simulink model "generic_src"  (Simulink 10.3)
settings: Solver=ode45  StartTime=0.0  StopTime=inf  RelTol=1e-3  EnableMultiTasking=on
undefined symbols (not defined in the file or in its folder): Area_Front, Area_Rear, ay_max_off, ay_max_on, ay_per_mu_max_off, ay_per_mu_max_on, Brake_ratio, brake_valve_ctrl_kP, cat1mode1_higher, cat1mode1_lower, cat1mode2_higher, cat1mode2_lower, cat1mode3_higher, cat1mode3_lower, cat2mode1_higher, cat2mode1_lower, cat2mode2_higher, cat2mode2_lower, cat2mode3_higher, cat2mode3_lower, delta_vel, diff_lock_fac, diff_lock_off, diff_lock_on, ESP_ctrl_kD, ESP_ctrl_kI, ESP_ctrl_kP, ESP_ctrl_restore_kI, ESP_min_throttle_fac, f_ax, f_slip, g, higherlimit_highvel, higherlimit_lowvel, highervel_fac, highervelocity_fac, InitialConditionForIntegrator, limit_acc, limit_selectlow, limit_starting, limit_vdiff, locktime_throttle, lowerlimit_highvel, lowerlimit_lowvel, lowervel_fac, lowervelocity_fac, min_throttle, MPS2KMPH, MSR_ctrl_kD, MSR_ctrl_kI, MSR_ctrl_kP, MSR_min_throttle_fac, PID_kP_sideslip, PID_kP_yawrate, RADpS2RpM, rBrake, RpM2RADpS, SH_SL_switch, sideslip_vel_corr, sidesplip_deviation_max ... (+35)
libraries: CarMaker4SL x136, simulink x55, simulink_extras x6
(part 1 of 9)
settings Model: Creator=IPG  LastModifiedBy=IPG  MultithreadedSim=on  ExtModeAutoUpdateStatusClock=off
settings DataIOCC: LimitDataPoints=on  SignalLoggingName=sigsOut
settings OptimizationCC: BooleanDataType=off  InitFltsAndDblsToZero=on
settings DebuggingCC: SaveWithParameterizedLinksMsg=none  SignalResolutionControl=TryResolveAllWithWarning  MultiTaskDSMMsg=warning  MultiTaskCondExecSysMsg=none  SFExecutionAtInitializationDiag=warning
settings HardwareCC: TargetUnknown=on
settings CodeAppCC: MaxIdLength=63
settings GRTTargetCC: TargetFcnLib=ansi_tfl_tmw.mat

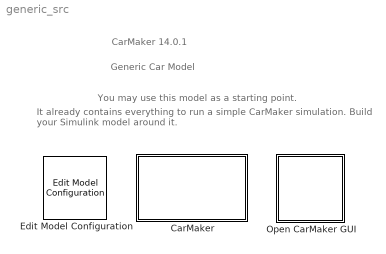
== system generic_src ==
  note: Generic Car Model
  note: You may use this model as a starting point.
  note: It already contains everything to run a simple CarMaker simulation.
      | Build your Simulink model around it.
  note: CarMaker 14.0.1
  CarMaker : Subsystem  TreatAsAtomicUnit=on
      mask Display: image(imread('CarMakerSys.png'));
  Edit Model Configuration : CarMaker4SL/Edit Model Configuration  SFunctionModules=''
  Open CarMaker GUI : Subsystem  LoadFcn=if ~length(which('cmself')), cmenv; end
      settings: OpenFcn=cmblockmagic('gui_fix_display'); CM_Simulink
      mask Display: image(imread('CarMakerGUI.png'));

== system generic_src/CarMaker ==
  CM_FIRST : Subsystem
  CM_LAST : Subsystem
  DrivMan : Subsystem
  Ground : Ground
  IPG Vehicle : Subsystem
  Terminator : Terminator
  VehicleControl : Subsystem
  wires:
  DrivMan/2(DrivMan.Out) -> VehicleControl/2(DrivMan.In)
  DrivMan/1(Sync_Out) -> VehicleControl/1(Sync_In)
  CM_FIRST/2(Env.Misc) -> DrivMan/2(Env.Misc)
  CM_FIRST/1(Sync_Out) -> DrivMan/1(Sync_In)
  CM_LAST/1(Sync_Out) -> Terminator/1
  Ground/1 -> CM_FIRST/1(Sync_In)
  IPG Vehicle/1(Sync_Out) -> CM_LAST/1(Sync_In)
  VehicleControl/1(Sync_Out) -> IPG Vehicle/1(Sync_In)
  VehicleControl/3(VhclCtrl.Steering) -> IPG Vehicle/3(VhclCtrl.Steering)
  VehicleControl/4(Vhcl.Wheel.In) -> IPG Vehicle/4(Vhcl.Wheel.In)
  VehicleControl/5(Vhcl.Misc) -> IPG Vehicle/5(Vhcl.Misc)
  VehicleControl/6(VhclCtrl.Brake) -> IPG Vehicle/6(VhclCtrl.Brake)
  VehicleControl/7(VhclCtrl.PT) -> IPG Vehicle/7(VhclCtrl.PT)
  VehicleControl/2(Vhcl.Model.Source) -> IPG Vehicle/2(Vhcl.Model.Source)

== system generic_src/Open CarMaker GUI ==
  S-Function : S-Function  FunctionName=cm_gui  SFunctionDeploymentMode=off  EnableBusSupport=off

== system generic_src/CarMaker/CM_FIRST ==
  Sync_In : Inport
  BusCreator1 : BusCreator  Inputs=8
  BusCreator2 : BusCreator  Inputs=6
  Demux1 : Demux  Outputs=14
      settings: DisplayOption=none
  Environment : S-Function  FunctionName=CM_Sfun  Parameters='Environment'  SFunctionDeploymentMode=off  EnableBusSupport=off
  IoIn : S-Function  FunctionName=CM_Sfun  Parameters='IoIn'  SFunctionDeploymentMode=off  EnableBusSupport=off
  Terminator : Terminator
  Sync_Out : Outport  VectorParamsAs1DForOutWhenUnconnected=off
  Env.Misc : Outport  Port=2  VectorParamsAs1DForOutWhenUnconnected=off
  wires:
  BusCreator2/1 -> Terminator/1  "IF Environment (in)"
  BusCreator1/1 -> Env.Misc/1
  Demux1/14 -> BusCreator2/6  "Env sRoad"
  Demux1/13 -> BusCreator2/5  "Env PoI_GCS Elev"
  Demux1/12 -> BusCreator2/4  "Env PoI_GCS Lat"
  Demux1/11 -> BusCreator2/3  "Env PoI_GCS Long"
  Demux1/10 -> BusCreator2/2  "Env Time"
  Demux1/9 -> BusCreator2/1  "Env yDay"
  Demux1/8 -> BusCreator1/8  "Env WindVel_tot z"
  Demux1/7 -> BusCreator1/7  "Env WindVel_tot y"
  Demux1/6 -> BusCreator1/6  "Env WindVel_tot x"
  Demux1/5 -> BusCreator1/5  "Env SolarRadiation"
  Demux1/4 -> BusCreator1/4  "Env AirHumidity"
  Demux1/3 -> BusCreator1/3  "Env AirPressure"
  Demux1/2 -> BusCreator1/2  "Env AirDensity"
  Demux1/1 -> BusCreator1/1  "Env Temperature"
  Environment/2 -> Demux1/1
  Environment/1 -> Sync_Out/1
  IoIn/1 -> Environment/1
  Sync_In/1 -> IoIn/1

== system generic_src/CarMaker/CM_LAST ==
  Sync_In : Inport
  CM_User : S-Function  FunctionName=CM_Sfun  Parameters='CM_User'  SFunctionDeploymentMode=off  EnableBusSupport=off
  IoOut : S-Function  FunctionName=CM_Sfun  Parameters='IoOut'  SFunctionDeploymentMode=off  EnableBusSupport=off
  Sync_Out : Outport  VectorParamsAs1DForOutWhenUnconnected=off
  wires:
  IoOut/1 -> Sync_Out/1
  CM_User/1 -> IoOut/1
  Sync_In/1 -> CM_User/1

== system generic_src/CarMaker/DrivMan ==
  note: There's rarely a reason to override DrivMan signals.
      | Use the VehicleControl interface for this purpose.
  Sync_In : Inport
  Env.Misc : Inport  Port=2
  BusCreator : BusCreator  Inputs=20
  Demux : Demux  Outputs=20
      settings: DisplayOption=none
  DrivMan : S-Function  FunctionName=CM_Sfun  Parameters='DrivMan'  SFunctionDeploymentMode=off  EnableBusSupport=off
  Ground : Ground
  Ground1 : Ground
  Ground2 : Ground
  Terminator : Terminator
  Terminator1 : Terminator
  Terminator2 : Terminator
  Sync_Out : Outport  VectorParamsAs1DForOutWhenUnconnected=off
  DrivMan.Out : Outport  Port=2  VectorParamsAs1DForOutWhenUnconnected=off
  wires:
  Demux/20 -> BusCreator/20  "DrivMan Steering Trq"
  Demux/19 -> BusCreator/19  "DrivMan Steering AngAcc"
  Demux/18 -> BusCreator/18  "DrivMan Steering AngVel"
  Demux/17 -> BusCreator/17  "DrivMan Steering Ang"
  Demux/16 -> BusCreator/16  "DrivMan Gas"
  Demux/15 -> BusCreator/15  "DrivMan Clutch"
  Demux/14 -> BusCreator/14  "DrivMan BrakePark"
  Demux/13 -> BusCreator/13  "DrivMan Brake"
  Demux/12 -> BusCreator/12  "DrivMan GearNo"
  Demux/8 -> BusCreator/8  "DrivMan SelectorCtrl"
  Demux/7 -> BusCreator/7  "DrivMan UserSignal4"
  Demux/6 -> BusCreator/6  "DrivMan UserSignal3"
  Demux/5 -> BusCreator/5  "DrivMan UserSignal2"
  Demux/4 -> BusCreator/4  "DrivMan UserSignal1"
  Demux/3 -> BusCreator/3  "DrivMan UserSignal0"
  Demux/2 -> BusCreator/2  "DrivMan Key"
  Env.Misc/1 -> DrivMan/2
  Sync_In/1 -> DrivMan/1
  DrivMan/1 -> Sync_Out/1
  BusCreator/1 -> DrivMan.Out/1
  DrivMan/2 -> Demux/1
  Demux/1 -> BusCreator/1  "DrivMan SST"
  Demux/9 -> Terminator/1  "DrivMan DigitalSelectorCtrl0"
  Demux/10 -> Terminator1/1  "DrivMan DigitalSelectorCtrl1"
  Demux/11 -> Terminator2/1  "DrivMan DigitalSelectorCtrl2"
  Ground/1 -> BusCreator/9
  Ground1/1 -> BusCreator/10
  Ground2/1 -> BusCreator/11

== system generic_src/CarMaker/IPG Vehicle ==
  Sync_In : Inport
  Vhcl.Model.Source : Inport  Port=2
  VhclCtrl.Steering : Inport  Port=3
  Vhcl.Wheel.In : Inport  Port=4
  Vhcl.Misc : Inport  Port=5
  VhclCtrl.Brake : Inport  Port=6
  VhclCtrl.PT : Inport  Port=7
  Brake : Subsystem
  CarAndTrailer : Subsystem
  PowerTrain : Subsystem
  Stop Simulation : Stop
  VehicleSource_BuiltIn : simulink/Logic and Bit Operations/Compare To Constant  relop=~=  const=1  OutDataTypeStr=boolean  ZeroCross=off
  Sync_Out : Outport  VectorParamsAs1DForOutWhenUnconnected=off
  wires:
  VhclCtrl.PT/1 -> PowerTrain/3(VhclCtrl.PT)
  Brake/1(Sync_Out) -> PowerTrain/1(Sync_In)
  CarAndTrailer/1(Sync_Out) -> Brake/1(Sync_In)
  CarAndTrailer/2(Brake.IF.In) -> Brake/2(Brake.IF.In)
  VhclCtrl.Brake/1 -> Brake/3(VhclCtrl.Brake)
  PowerTrain/1(Sync_Out) -> Sync_Out/1
  Vhcl.Misc/1 -> CarAndTrailer/4(Vhcl.Misc)
  Vhcl.Wheel.In/1 -> CarAndTrailer/3(Vhcl.Wheel.In)
  VhclCtrl.Steering/1 -> CarAndTrailer/2(VhclCtrl.Steering)
  Sync_In/1 -> CarAndTrailer/1(Sync_In)
  Vhcl.Model.Source/1 -> VehicleSource_BuiltIn/1
  VehicleSource_BuiltIn/1 -> Stop Simulation/1
  Brake/2(Vhcl.Wheel.PT) -> PowerTrain/2(Vhcl.Wheel.PT)

== system generic_src/CarMaker/VehicleControl ==
  note: <Your model here>
  note: When implementing a vehicle control model,
      | be sure to add '-disablevehiclecontrol' to the command line arguments
      | in the CarMaker Model Configuration block.
      | Otherwise your model will possibly not see the original DrivMan signals
      | on its inputs, but those of a currently activated C-coded vehicle control model instead.
  Sync_In : Inport
  DrivMan.In : Inport  Port=2
  Bus Creator2 : BusCreator  Inputs=2
  CreateBus Vhcl.Misc : Subsystem
  CreateBus Vhcl.Wheel.In : Subsystem
  CreateBus VhclCtrl : Subsystem
  CreateBus VhclCtrl.PT : Subsystem
  CreateBus VhclCtrl.Steering : Subsystem
  Demux2 : Demux  Outputs=2
      settings: DisplayOption=none
  VehicleControl : S-Function  FunctionName=CM_Sfun  Parameters='VehicleControl'  SFunctionDeploymentMode=off  EnableBusSupport=off
  VehicleControlUpd : S-Function  FunctionName=CM_Sfun  Parameters='VehicleControlUpd'  SFunctionDeploymentMode=off  EnableBusSupport=off
  Sync_Out : Outport  VectorParamsAs1DForOutWhenUnconnected=off
  Vhcl.Model.Source : Outport  Port=2  VectorParamsAs1DForOutWhenUnconnected=off
  VhclCtrl.Steering : Outport  Port=3  VectorParamsAs1DForOutWhenUnconnected=off
  Vhcl.Wheel.In : Outport  Port=4  VectorParamsAs1DForOutWhenUnconnected=off
  Vhcl.Misc : Outport  Port=5  VectorParamsAs1DForOutWhenUnconnected=off
  VhclCtrl.Brake : Outport  Port=6  VectorParamsAs1DForOutWhenUnconnected=off
  VhclCtrl.PT : Outport  Port=7  VectorParamsAs1DForOutWhenUnconnected=off
  wires:
  CreateBus VhclCtrl/1(Out) -> VehicleControlUpd/2
  VehicleControl/2 -> CreateBus VhclCtrl/1(In)
  VehicleControlUpd/2 -> Vhcl.Model.Source/1
  VehicleControlUpd/4 -> CreateBus Vhcl.Wheel.In/1(In1)
  VehicleControlUpd/5 -> CreateBus Vhcl.Misc/1(In1)
  VehicleControlUpd/6 -> Demux2/1
  VehicleControlUpd/7 -> CreateBus VhclCtrl.PT/1(In1)
  VehicleControlUpd/3 -> CreateBus VhclCtrl.Steering/1(In1)
  CreateBus Vhcl.Misc/1(Out1) -> Vhcl.Misc/1
  CreateBus Vhcl.Wheel.In/1(Out1) -> Vhcl.Wheel.In/1
  DrivMan.In/1 -> VehicleControl/2
  VehicleControl/1 -> VehicleControlUpd/1
  Sync_In/1 -> VehicleControl/1
  CreateBus VhclCtrl.PT/1(Out1) -> VhclCtrl.PT/1
  Bus Creator2/1 -> VhclCtrl.Brake/1
  CreateBus VhclCtrl.Steering/1(Out1) -> VhclCtrl.Steering/1
  VehicleControlUpd/1 -> Sync_Out/1
  Demux2/2 -> Bus Creator2/2  "VhclCtrl BrakePark"
  Demux2/1 -> Bus Creator2/1  "VhclCtrl Brake"

== system generic_src/CarMaker/IPG Vehicle/Brake ==
  note: When replacing the entire braking system,
      | be sure to disable the IPG brake model by using the brake
      | model 'Model Manager off' in the vehicle GUI.
  note: <Your model here>
  Sync_In : Inport
  Brake.IF.In : Inport  Port=2
  VhclCtrl.Brake : Inport  Port=3
  Brake : S-Function  FunctionName=CM_Sfun  Parameters='Brake'  SFunctionDeploymentMode=off  EnableBusSupport=off
  BrakeUpd : S-Function  FunctionName=CM_Sfun  Parameters='BrakeUpd'  SFunctionDeploymentMode=off  EnableBusSupport=off
  BusCreator1 : BusCreator  Inputs=16
  CreateBus Vhcl.Wheel.PT : Subsystem
  Demux : Demux  Outputs=16
      settings: DisplayOption=none
  HydBrakeCU Example : Subsystem
  Sync_Out : Outport  VectorParamsAs1DForOutWhenUnconnected=off
  Vhcl.Wheel.PT : Outport  Port=2  VectorParamsAs1DForOutWhenUnconnected=off
  wires:
  Demux/16 -> BusCreator1/16  "Brake IF Trq_DriveSrc_trg d3"
  Demux/15 -> BusCreator1/15  "Brake IF Trq_DriveSrc_trg d2"
  Demux/14 -> BusCreator1/14  "Brake IF Trq_DriveSrc_trg d1"
  Demux/13 -> BusCreator1/13  "Brake IF Trq_DriveSrc_trg d0"
  Demux/12 -> BusCreator1/12  "Brake IF Trq_Reg_trg RR"
  Demux/11 -> BusCreator1/11  "Brake IF Trq_Reg_trg RL"
  Demux/10 -> BusCreator1/10  "Brake IF Trq_Reg_trg FR"
  Demux/9 -> BusCreator1/9  "Brake IF Trq_Reg_trg FL"
  Demux/8 -> BusCreator1/8  "Brake IF Trq_PB RR"
  Demux/7 -> BusCreator1/7  "Brake IF Trq_PB RL"
  Demux/6 -> BusCreator1/6  "Brake IF Trq_PB FR"
  Demux/5 -> BusCreator1/5  "Brake IF Trq_PB FL"
  Demux/4 -> BusCreator1/4  "Brake IF Trq_WB RR"
  Demux/3 -> BusCreator1/3  "Brake IF Trq_WB RL"
  Demux/2 -> BusCreator1/2  "Brake IF Trq_WB FR"
  Demux/1 -> BusCreator1/1  "Brake IF Trq_WB FL"
  Brake/2 -> Demux/1
  BusCreator1/1 -> BrakeUpd/2
  BrakeUpd/1 -> Sync_Out/1
  Brake/1 -> BrakeUpd/1  "Sync"
  Brake.IF.In/1 -> Brake/2
  VhclCtrl.Brake/1 -> Brake/3
  Sync_In/1 -> Brake/1
  BrakeUpd/2 -> CreateBus Vhcl.Wheel.PT/1(In)
  CreateBus Vhcl.Wheel.PT/1(Out) -> Vhcl.Wheel.PT/1

== system generic_src/CarMaker/IPG Vehicle/CarAndTrailer ==
  Sync_In : Inport
  VhclCtrl.Steering : Inport  Port=2
  Vhcl.Wheel.In : Inport  Port=3
  Vhcl.Misc : Inport  Port=4
  CarAndTrailerUpd : Subsystem
  Forces : Subsystem
  Ground : Ground
  Kinematics : Subsystem
  Kinetics : Subsystem
  Steering : Subsystem
  Terminator : Terminator
  Terminator1 : Terminator
  Trailer : Subsystem
  Sync_Out : Outport  VectorParamsAs1DForOutWhenUnconnected=off
  Brake.IF.In : Outport  Port=2  VectorParamsAs1DForOutWhenUnconnected=off
  wires:
  Trailer/9(Car.Hitch.FrcTrq) -> CarAndTrailerUpd/9(Car.Hitch.FrcTrq)
  Trailer/8(Vhcl.Wheel.RR) -> CarAndTrailerUpd/8(Vhcl.Wheel.RR)
  Trailer/7(Vhcl.Wheel.RL) -> CarAndTrailerUpd/7(Vhcl.Wheel.RL)
  Trailer/6(Vhcl.Wheel.FR) -> CarAndTrailerUpd/6(Vhcl.Wheel.FR)
  Trailer/5(Vhcl.Wheel.FL) -> CarAndTrailerUpd/5(Vhcl.Wheel.FL)
  Trailer/4(Vhcl.PoI) -> CarAndTrailerUpd/4(Vhcl.PoI)
  Trailer/3(Vhcl.Motion) -> CarAndTrailerUpd/3(Vhcl.Motion)
  Trailer/2(Vhcl.Steering) -> CarAndTrailerUpd/2(Vhcl.Steering)
  Trailer/1(Sync_Out) -> CarAndTrailerUpd/1(Sync_In)
  CarAndTrailerUpd/2(Brake.IF.In) -> Brake.IF.In/1
  CarAndTrailerUpd/1(Sync_Out) -> Sync_Out/1
  Vhcl.Misc/1 -> Terminator1/1
  Vhcl.Wheel.In/1 -> Terminator/1
  Kinetics/6(WheelCarrier.Misc) -> Trailer/6(WheelCarrier.Misc)
  Kinetics/5(Car.Trq_T2W) -> Trailer/5(Car.Trq_T2W)
  Steering/2(Steer.IF) -> ?
  Kinetics/4(Car.Fr1) -> Trailer/4(Car.Fr1)
  Kinetics/3(Car.Hitch) -> Trailer/3(Car.Hitch)
  Kinetics/2(Trailer.Load) -> Trailer/2(Trailer.Load)
  VhclCtrl.Steering/1 -> Steering/2(VhclCtrl.Steering)
  Sync_In/1 -> Steering/1(Sync_In)
  Steering/1(Sync_Out) -> ?
  Kinetics/1(Sync_Out) -> Trailer/1(Sync_In)
  Ground/1 -> CarAndTrailerUpd/10(Vhcl.Fr1A)
  ? -> ?
  ? -> ?
  ? -> ?
  Forces/8(TireRR_Out) -> ?
  Forces/7(TireRL_Out) -> ?
  Forces/6(TireFR_Out) -> ?
  Forces/5(TireFL_Out) -> ?
  Forces/4(Car.Load) -> ?
  Forces/2(Car.Virtual) -> ?
  ? -> Forces/6(lSpring)
  ? -> Forces/7(vDamp)
  Forces/3(Car.Aero) -> ?
  Forces/1(Sync_Out) -> ?
  ? -> Forces/5(TireRR_In)
  ? -> Forces/4(TireRL_In)
  ? -> Forces/3(TireFR_In)
  ? -> Forces/2(TireFL_In)
  ? -> Forces/1(Sync_In)
  ? -> Forces/8(lStabi)
  ? -> ?
  ? -> Forces/9(lBuf)

== system generic_src/CarMaker/IPG Vehicle/PowerTrain ==
  note: When replacing the entire powertrain,
      | be sure to disable the IPG powertrain model by using the powertrain
      | model 'Model Manager off' in the vehicle GUI.
  note: <Your model here>
  Sync_In : Inport
  Vhcl.Wheel.PT : Inport  Port=2
  VhclCtrl.PT : Inport  Port=3
  BusCreator1 : BusCreator  Inputs=42
  Demux1 : Demux  Outputs=42
      settings: DisplayOption=none
  Ground : Ground
  MCU Example : Subsystem
  PTControl Example : Subsystem
  PowerTrain : S-Function  FunctionName=CM_Sfun  Parameters='PowerTrain'  SFunctionDeploymentMode=off  EnableBusSupport=off
  PowerTrainUpd : S-Function  FunctionName=CM_Sfun  Parameters='PowerTrainUpd'  SFunctionDeploymentMode=off  EnableBusSupport=off
  Sync_Out : Outport  VectorParamsAs1DForOutWhenUnconnected=off
  wires:
  BusCreator1/1 -> PowerTrainUpd/2
  Demux1/42 -> BusCreator1/42  "PT IF WRR Trq_BrakeReg_max"
  Demux1/41 -> BusCreator1/41  "PT IF WRR Trq_BrakeReg"
  Demux1/40 -> BusCreator1/40  "PT IF WRR Trq_Supp2WC"
  Demux1/39 -> BusCreator1/39  "PT IF WRR Trq_Drive"
  Demux1/38 -> BusCreator1/38  "PT IF WRR Trq_B2W"
  Demux1/37 -> BusCreator1/37  "PT IF WRR rotv"
  Demux1/36 -> BusCreator1/36  "PT IF WRR rot"
  Demux1/35 -> BusCreator1/35  "PT IF WRL Trq_BrakeReg_max"
  Demux1/34 -> BusCreator1/34  "PT IF WRL Trq_BrakeReg"
  Demux1/33 -> BusCreator1/33  "PT IF WRL Trq_Supp2WC"
  Demux1/32 -> BusCreator1/32  "PT IF WRL Trq_Drive"
  Demux1/31 -> BusCreator1/31  "PT IF WRL Trq_B2W"
  Demux1/30 -> BusCreator1/30  "PT IF WRL rotv"
  Demux1/29 -> BusCreator1/29  "PT IF WRL rot"
  Demux1/28 -> BusCreator1/28  "PT IF WFR Trq_BrakeReg_max"
  Demux1/27 -> BusCreator1/27  "PT IF WFR Trq_BrakeReg"
  Demux1/26 -> BusCreator1/26  "PT IF WFR Trq_Supp2WC"
  Demux1/25 -> BusCreator1/25  "PT IF WFR Trq_Drive"
  Demux1/24 -> BusCreator1/24  "PT IF WFR Trq_B2W"
  Demux1/23 -> BusCreator1/23  "PT IF WFR rotv"
  Demux1/22 -> BusCreator1/22  "PT IF WFR rot"
  Demux1/21 -> BusCreator1/21  "PT IF WFL Trq_BrakeReg_max"
  Demux1/20 -> BusCreator1/20  "PT IF WFL Trq_BrakeReg"
  Demux1/19 -> BusCreator1/19  "PT IF WFL Trq_Supp2WC"
  Demux1/18 -> BusCreator1/18  "PT IF WFL Trq_Drive"
  Demux1/17 -> BusCreator1/17  "PT IF WFL Trq_B2W"
  Demux1/16 -> BusCreator1/16  "PT IF WFL rotv"
  Demux1/15 -> BusCreator1/15  "PT IF WFL rot"
  Demux1/14 -> BusCreator1/14  "PT IF DL_iDiff_mean"
  Demux1/13 -> BusCreator1/13  "PT IF Trq_Supp2BdyEng y"
  Demux1/12 -> BusCreator1/12  "PT IF Trq_Supp2BdyEng x"
  Demux1/11 -> BusCreator1/11  "PT IF Trq_Supp2Bdy1B z"
  Demux1/10 -> BusCreator1/10  "PT IF Trq_Supp2Bdy1B y"
  Demux1/9 -> BusCreator1/9  "PT IF Trq_Supp2Bdy1B x"
  Demux1/8 -> BusCreator1/8  "PT IF Trq_Supp2Bdy1 z"
  Demux1/7 -> BusCreator1/7  "PT IF Trq_Supp2Bdy1 y"
  Demux1/6 -> BusCreator1/6  "PT IF Trq_Supp2Bdy1 x"
  Demux1/5 -> BusCreator1/5  "PT IF Engine_rotv"
  Demux1/4 -> BusCreator1/4  "PT IF GearNo"
  Demux1/3 -> BusCreator1/3  "PT IF OperationError"
  Demux1/2 -> BusCreator1/2  "PT IF OperationState"
  Demux1/1 -> BusCreator1/1  "PT IF Ignition"
  Sync_In/1 -> PowerTrain/1
  PowerTrain/2 -> Demux1/1
  PowerTrainUpd/1 -> Sync_Out/1
  PowerTrain/1 -> PowerTrainUpd/1  "Sync"
  VhclCtrl.PT/1 -> PowerTrain/3
  Vhcl.Wheel.PT/1 -> PowerTrain/2
  Ground/1 -> PTControl Example/1(Sync_In), MCU Example/1(Sync_In), PTControl Example/2(VhclCtrl.PT)

== system generic_src/CarMaker/VehicleControl/CreateBus Vhcl.Misc ==
  In1 : Inport
  BusCreator : BusCreator  Inputs=11
  Demux : Demux  Outputs=11
      settings: DisplayOption=none
  Out1 : Outport  VectorParamsAs1DForOutWhenUnconnected=off
  wires:
  Demux/11 -> BusCreator/11  "Vhcl Wind_vel_0 z"
  Demux/10 -> BusCreator/10  "Vhcl Wind_vel_0 y"
  Demux/9 -> BusCreator/9  "Vhcl Wind_vel_0 x"
  Demux/8 -> BusCreator/8  "Vhcl Trq_DL2BdyEng y"
  Demux/7 -> BusCreator/7  "Vhcl Trq_DL2BdyEng x"
  Demux/6 -> BusCreator/6  "Vhcl Trq_DL2Bdy1B z"
  Demux/5 -> BusCreator/5  "Vhcl Trq_DL2Bdy1B y"
  Demux/4 -> BusCreator/4  "Vhcl Trq_DL2Bdy1B x"
  Demux/3 -> BusCreator/3  "Vhcl Trq_DL2Bdy1 z"
  Demux/2 -> BusCreator/2  "Vhcl Trq_DL2Bdy1 y"
  Demux/1 -> BusCreator/1  "Vhcl Trq_DL2Bdy1 x"
  In1/1 -> Demux/1
  BusCreator/1 -> Out1/1

== system generic_src/CarMaker/VehicleControl/CreateBus Vhcl.Wheel.In ==
  In1 : Inport
  Bus Creator1 : BusCreator  Inputs=12
  Demux1 : Demux  Outputs=12
      settings: DisplayOption=none
  Out1 : Outport  VectorParamsAs1DForOutWhenUnconnected=off
  wires:
  Demux1/12 -> Bus Creator1/12  "Vhcl Wheel RR rotv"
  Demux1/11 -> Bus Creator1/11  "Vhcl Wheel RR Trq_DL2WC"
  Demux1/10 -> Bus Creator1/10  "Vhcl Wheel RR Trq_B2WC"
  Demux1/9 -> Bus Creator1/9  "Vhcl Wheel RL rotv"
  Demux1/8 -> Bus Creator1/8  "Vhcl Wheel RL Trq_DL2WC"
  Demux1/7 -> Bus Creator1/7  "Vhcl Wheel RL Trq_B2WC"
  Demux1/6 -> Bus Creator1/6  "Vhcl Wheel FR rotv"
  Demux1/5 -> Bus Creator1/5  "Vhcl Wheel FR Trq_DL2WC"
  Demux1/4 -> Bus Creator1/4  "Vhcl Wheel FR Trq_B2WC"
  Demux1/3 -> Bus Creator1/3  "Vhcl Wheel FL rotv"
  In1/1 -> Demux1/1
  Bus Creator1/1 -> Out1/1
  Demux1/2 -> Bus Creator1/2  "Vhcl Wheel FL Trq_DL2WC"
  Demux1/1 -> Bus Creator1/1  "Vhcl Wheel FL Trq_B2WC"

== system generic_src/CarMaker/VehicleControl/CreateBus VhclCtrl ==
  In : Inport
  BusCreator : BusCreator  Inputs=29
  Demux : Demux  Outputs=29
      settings: DisplayOption=none
  Out : Outport  VectorParamsAs1DForOutWhenUnconnected=off
  wires:
  In/1 -> Demux/1
  BusCreator/1 -> Out/1
  Demux/1 -> BusCreator/1  "VhclCtrl SST"
  Demux/2 -> BusCreator/2  "VhclCtrl Key"
  Demux/3 -> BusCreator/3  "VhclCtrl UserSignal0"
  Demux/4 -> BusCreator/4  "VhclCtrl UserSignal1"
  Demux/5 -> BusCreator/5  "VhclCtrl UserSignal2"
  Demux/6 -> BusCreator/6  "VhclCtrl UserSignal3"
  Demux/7 -> BusCreator/7  "VhclCtrl UserSignal4"
  Demux/8 -> BusCreator/8  "VhclCtrl GearNo"
  Demux/9 -> BusCreator/9  "VhclCtrl SelectorCtrl"
  Demux/10 -> BusCreator/10  "VhclCtrl Brake"
  Demux/11 -> BusCreator/11  "VhclCtrl BrakePark"
  Demux/12 -> BusCreator/12  "VhclCtrl Clutch"
  Demux/13 -> BusCreator/13  "VhclCtrl Gas"
  Demux/14 -> BusCreator/14  "VhclCtrl Steering Ang"
  Demux/15 -> BusCreator/15  "VhclCtrl Steering AngVel"
  Demux/16 -> BusCreator/16  "VhclCtrl Steering AngAcc"
  Demux/17 -> BusCreator/17  "VhclCtrl Steering Trq"
  Demux/18 -> BusCreator/18  "VhclCtrl Lights LowBeam"
  Demux/19 -> BusCreator/19  "VhclCtrl Lights HighBeam"
  Demux/20 -> BusCreator/20  "VhclCtrl Lights Daytime"
  Demux/21 -> BusCreator/21  "VhclCtrl Lights ParkL"
  Demux/22 -> BusCreator/22  "VhclCtrl Lights ParkR"
  Demux/23 -> BusCreator/23  "VhclCtrl Lights IndL"
  Demux/24 -> BusCreator/24  "VhclCtrl Lights IndR"
  Demux/25 -> BusCreator/25  "VhclCtrl Lights FogFrontL"
  Demux/26 -> BusCreator/26  "VhclCtrl Lights FogFrontR"
  Demux/27 -> BusCreator/27  "VhclCtrl Lights FogRear"
  Demux/28 -> BusCreator/28  "VhclCtrl Lights Brake"
  Demux/29 -> BusCreator/29  "VhclCtrl Lights Reverse"

== system generic_src/CarMaker/VehicleControl/CreateBus VhclCtrl.PT ==
  In1 : Inport
  BusCreator1 : BusCreator  Inputs=12
  Demux1 : Demux  Outputs=12
      settings: DisplayOption=none
  Out1 : Outport  VectorParamsAs1DForOutWhenUnconnected=off
  wires:
  Demux1/12 -> BusCreator1/12  "VhclCtrl Brake"
  Demux1/11 -> BusCreator1/11  "VhclCtrl Gas"
  Demux1/10 -> BusCreator1/10  "VhclCtrl Clutch"
  Demux1/9 -> BusCreator1/9  "VhclCtrl SelectorCtrl"
  Demux1/8 -> BusCreator1/8  "VhclCtrl GearNo"
  Demux1/7 -> BusCreator1/7  "VhclCtrl UserSignal4"
  Demux1/6 -> BusCreator1/6  "VhclCtrl UserSignal3"
  Demux1/5 -> BusCreator1/5  "VhclCtrl UserSignal2"
  Demux1/4 -> BusCreator1/4  "VhclCtrl UserSignal1"
  Demux1/3 -> BusCreator1/3  "VhclCtrl UserSignal0"
  Demux1/2 -> BusCreator1/2  "VhclCtrl Key"
  Demux1/1 -> BusCreator1/1  "VhclCtrl SST"
  In1/1 -> Demux1/1
  BusCreator1/1 -> Out1/1

== system generic_src/CarMaker/VehicleControl/CreateBus VhclCtrl.Steering ==
  In1 : Inport
  Bus Creator : BusCreator  Inputs=5
  Demux : Demux  Outputs=5
      settings: DisplayOption=none
  Out1 : Outport  VectorParamsAs1DForOutWhenUnconnected=off
  wires:
  In1/1 -> Demux/1
  Bus Creator/1 -> Out1/1
  Demux/1 -> Bus Creator/1  "VhclCtrl Steering Ang"
  Demux/5 -> Bus Creator/5  "VhclCtrl Steering SteerByTrq"
  Demux/3 -> Bus Creator/3  "VhclCtrl Steering AngAcc"
  Demux/2 -> Bus Creator/2  "VhclCtrl Steering AngVel"
  Demux/4 -> Bus Creator/4  "VhclCtrl Steering Trq"

== system generic_src/CarMaker/IPG Vehicle/Brake/CreateBus Vhcl.Wheel.PT ==
  In : Inport
  BusCreator1 : BusCreator  Inputs=20
  Demux1 : Demux  Outputs=20
      settings: DisplayOption=none
  Out : Outport  VectorParamsAs1DForOutWhenUnconnected=off
  wires:
  Demux1/20 -> BusCreator1/20  "Vhcl Trq_DriveSrc_trg d3"
  Demux1/19 -> BusCreator1/19  "Vhcl Trq_DriveSrc_trg d2"
  Demux1/18 -> BusCreator1/18  "Vhcl Trq_DriveSrc_trg d1"
  Demux1/17 -> BusCreator1/17  "Vhcl Trq_DriveSrc_trg d0"
  Demux1/16 -> BusCreator1/16  "Vhcl Wheel RR WhlBearing"
  Demux1/15 -> BusCreator1/15  "Vhcl Wheel RR Trq_T2W"
  Demux1/14 -> BusCreator1/14  "Vhcl Wheel RR Trq_BrakeReg_trg"
  Demux1/13 -> BusCreator1/13  "Vhcl Wheel RR Trq_Brake"
  Demux1/12 -> BusCreator1/12  "Vhcl Wheel RL WhlBearing"
  Demux1/11 -> BusCreator1/11  "Vhcl Wheel RL Trq_T2W"
  Demux1/10 -> BusCreator1/10  "Vhcl Wheel RL Trq_BrakeReg_trg"
  Demux1/9 -> BusCreator1/9  "Vhcl Wheel RL Trq_Brake"
  Demux1/8 -> BusCreator1/8  "Vhcl Wheel FR WhlBearing"
  Demux1/7 -> BusCreator1/7  "Vhcl Wheel FR Trq_T2W"
  Demux1/6 -> BusCreator1/6  "Vhcl Wheel FR Trq_BrakeReg_trg"
  Demux1/5 -> BusCreator1/5  "Vhcl Wheel FR Trq_Brake"
  Demux1/4 -> BusCreator1/4  "Vhcl Wheel FL WhlBearing"
  Demux1/3 -> BusCreator1/3  "Vhcl Wheel FL Trq_T2W"
  Demux1/2 -> BusCreator1/2  "Vhcl Wheel FL Trq_BrakeReg_trg"
  Demux1/1 -> BusCreator1/1  "Vhcl Wheel FL Trq_Brake"
  BusCreator1/1 -> Out/1
  In/1 -> Demux1/1

== system generic_src/CarMaker/IPG Vehicle/Brake/HydBrakeCU Example ==
  Sync_In : Inport
  Bus Assignment : BusAssignment  AssignedSignals=HydBrakeCU_Out Valve_FL_Inlet,HydBrakeCU_Out Valve_FR_Inlet,HydBrakeCU_Out Valve_RL_Inlet,HydBrakeCU_Out Valve_RR_Inlet,HydBrakeCU_Out Valve_FL_Outlet,HydBrakeCU_Out Valve_FR_Outlet,HydBrakeCU_Out Valve_RL_Outlet,HydBrakeCU_Out Valve_RR_Outlet,HydBrakeCU_Out Valve_PV_1,HydBrakeCU_Out Valve_PV_2,HydBrakeCU_Out Valve_SV_1,HydBrakeCU_Out Valve_SV_2,HydBrakeCU_Out PumpCtrl,HydBrakeCU_Out Park,HydBrakeCU_Out Pedal,HydBrakeCU_Out Trq_DriveSrc_trg_d0,HydBrakeCU_Out Trq_DriveSrc_trg_d1,HydBrakeCU_Out Trq_DriveSrc_trg_d2,HydBrakeCU_Out Trq_DriveSrc_trg_d3
  Bus Creator : BusCreator  Inputs=30
  Bus Selector : BusSelector  OutputSignals=HydBrakeCU.HydBrakeCU Pedal,HydBrakeCU.HydBrakeCU Park,HydBrakeCU.HydBrakeCU Trq_BrakeReg_max_FL,HydBrakeCU.HydBrakeCU Trq_BrakeReg_max_FR,HydBrakeCU.HydBrakeCU Trq_BrakeReg_max_RL,HydBrakeCU.HydBrakeCU Trq_BrakeReg_max_RR,HydBrakeCU.HydBrakeCU Trq_BrakeReg_FL,HydBrakeCU.HydBrakeCU Trq_BrakeReg_FR,HydBrakeCU.HydBrakeCU Trq_BrakeReg_RL,HydBrakeCU.HydBrakeCU Trq_BrakeReg_RR,HydBrakeCU.HydBrakeCU T_env,HydBrakeCU.HydBrakeCU Trq_WB_FL,HydBrakeCU.HydBrakeCU Trq_WB_FR,HydBrakeCU.HydBrakeCU Trq_WB_RL,HydBrakeCU.HydBrakeCU Trq_WB_RR,HydBrakeCU.HydBrakeCU Trq_PB_FL,HydBrakeCU.HydBrakeCU Trq_PB_FR,HydBrakeCU.HydBrakeCU Trq_PB_RL,HydBrakeCU.HydBrakeCU Trq_PB_RR,HydBrakeCU.HydBrakeCU Rel_SW,HydBrakeCU.HydBrakeCU pMC,HydBrakeCU.HydBrakeCU pWB_FL,HydBrakeCU.HydBrakeCU pWB_FR,HydBrakeCU.HydBrakeCU pWB_RL,HydBrakeCU.HydBrakeCU pWB_RR,HydBrakeCU.HydBrakeCU PuRetVolt,HydBrakeCU.HydBrakeCU PedFrc,HydBrakeCU.HydBrakeCU PedTravel,HydBrakeCU.HydBrakeCU PistTravel,HydBrakeCU.HydBrakeCU DiaphTravel
  Bus Selector2 : BusSelector  OutputSignals=Brake Valves.Valve_In_FL,Brake Valves.Valve_In_FR,Brake Valves.Valve_In_RL,Brake Valves.Valve_In_RR,Brake Valves.Valve_Out_FL,Brake Valves.Valve_Out_FR,Brake Valves.Valve_Out_RL,Brake Valves.Valve_Out_RR,Pilot Valves.Valve_PV_0,Pilot Valves.Valve_PV_1,Suction Valves.Valve_SV_0,Suction Valves.Valve_SV_1,Pump Ctrl,BrakePark,Brake Pedal Position
  Compare To Constant : simulink/Logic and Bit Operations/Compare To Constant  relop===  const=8  OutDataTypeStr=uint8
  Constant : Constant  Value=-99999
  CreateBus HydBrakeCU : Subsystem
  ESP Controller : Subsystem  TreatAsAtomicUnit=on
  Ground PTC WheelOut : Ground
  HydBrakeCtrl_In : Subsystem
  HydBrakeCtrl_Out : Subsystem
  Read CM Dict : CarMaker4SL/Read CM Dict  xname=SC.State  xsync=off  xstime=Continuous
  wires:
  Sync_In/1 -> HydBrakeCtrl_In/1(Sync_In)
  HydBrakeCtrl_In/1(HydBrakeCtrl_In) -> Bus Selector/1
  Ground PTC WheelOut/1 -> CreateBus HydBrakeCU/1(In)
  CreateBus HydBrakeCU/1(Out) -> Bus Assignment/1
  Bus Creator/1 -> ESP Controller/1(HydBrakeCtrl_In)
  Bus Selector/1 -> Bus Creator/1  "<HydBrakeCU Pedal>"
  Bus Selector/2 -> Bus Creator/2  "<HydBrakeCU Park>"
  Bus Selector/3 -> Bus Creator/3  "<HydBrakeCU Trq_BrakeReg_max_FL>"
  Bus Selector/4 -> Bus Creator/4  "<HydBrakeCU Trq_BrakeReg_max_FR>"
  Bus Selector/5 -> Bus Creator/5  "<HydBrakeCU Trq_BrakeReg_max_RL>"
  Bus Selector/6 -> Bus Creator/6  "<HydBrakeCU Trq_BrakeReg_max_RR>"
  Bus Selector/7 -> Bus Creator/7  "<HydBrakeCU Trq_BrakeReg_FL>"
  Bus Selector/8 -> Bus Creator/8  "<HydBrakeCU Trq_BrakeReg_FR>"
  Bus Selector/9 -> Bus Creator/9  "<HydBrakeCU Trq_BrakeReg_RL>"
  Bus Selector/10 -> Bus Creator/10  "<HydBrakeCU Trq_BrakeReg_RR>"
  Bus Selector/11 -> Bus Creator/11  "<HydBrakeCU T_env>"
  Bus Selector/12 -> Bus Creator/12  "<HydBrakeCU Trq_WB_FL>"
  Bus Selector/13 -> Bus Creator/13  "<HydBrakeCU Trq_WB_FR>"
  Bus Selector/14 -> Bus Creator/14  "<HydBrakeCU Trq_WB_RL>"
  Bus Selector/15 -> Bus Creator/15  "<HydBrakeCU Trq_WB_RR>"
  Bus Selector/16 -> Bus Creator/16  "<HydBrakeCU Trq_PB_FL>"
  Bus Selector/17 -> Bus Creator/17  "<HydBrakeCU Trq_PB_FR>"
  Bus Selector/18 -> Bus Creator/18  "<HydBrakeCU Trq_PB_RL>"
  Bus Selector/19 -> Bus Creator/19  "<HydBrakeCU Trq_PB_RR>"
  Bus Selector/20 -> Bus Creator/20  "<HydBrakeCU Rel_SW>"
  Bus Selector/21 -> Bus Creator/21  "<HydBrakeCU pMC>"
  Bus Selector/22 -> Bus Creator/22  "<HydBrakeCU pWB_FL>"
  Bus Selector/23 -> Bus Creator/23  "<HydBrakeCU pWB_FR>"
  Bus Selector/24 -> Bus Creator/24  "<HydBrakeCU pWB_RL>"
  Bus Selector/25 -> Bus Creator/25  "<HydBrakeCU pWB_RR>"
  Bus Selector/26 -> Bus Creator/26  "<HydBrakeCU PuRetVolt>"
  Bus Selector/27 -> Bus Creator/27  "<HydBrakeCU PedFrc>"
  Bus Selector/28 -> Bus Creator/28  "<HydBrakeCU PedTravel>"
  Bus Selector/29 -> Bus Creator/29  "<HydBrakeCU PistTravel>"
  Bus Selector/30 -> Bus Creator/30  "<HydBrakeCU DiaphTravel>"
  ESP Controller/1(HydBrakeCU_Out) -> Bus Selector2/1
  Bus Selector2/1 -> Bus Assignment/2  "<Valve_In_FL>"
  Bus Selector2/2 -> Bus Assignment/3  "<Valve_In_FR>"
  Bus Selector2/3 -> Bus Assignment/4  "<Valve_In_RL>"
  Bus Selector2/4 -> Bus Assignment/5  "<Valve_In_RR>"
  Bus Selector2/5 -> Bus Assignment/6  "<Valve_Out_FL>"
  Bus Selector2/6 -> Bus Assignment/7  "<Valve_Out_FR>"
  Bus Selector2/7 -> Bus Assignment/8  "<Valve_Out_RL>"
  Bus Selector2/8 -> Bus Assignment/9  "<Valve_Out_RR>"
  Bus Selector2/9 -> Bus Assignment/10  "<Valve_PV_0>"
  Bus Selector2/10 -> Bus Assignment/11  "<Valve_PV_1>"
  Bus Selector2/11 -> Bus Assignment/12  "<Valve_SV_0>"
  Bus Selector2/12 -> Bus Assignment/13  "<Valve_SV_1>"
  Bus Selector2/13 -> Bus Assignment/14  "<Pump Ctrl>"
  Bus Selector2/14 -> Bus Assignment/15  "<BrakePark>"
  Bus Assignment/1 -> HydBrakeCtrl_Out/1(HydBrakeCU)
  Read CM Dict/1 -> Compare To Constant/1
  Compare To Constant/1 -> ESP Controller/Enable
  Bus Selector2/15 -> Bus Assignment/16  "<Brake Pedal Position>"
  Constant/1 -> Bus Assignment/20, Bus Assignment/19, Bus Assignment/18, Bus Assignment/17

== system generic_src/CarMaker/IPG Vehicle/CarAndTrailer/CarAndTrailerUpd ==
  Sync_In : Inport
  Vhcl.Steering : Inport  Port=2
  Vhcl.Motion : Inport  Port=3
  Vhcl.PoI : Inport  Port=4
  Vhcl.Wheel.FL : Inport  Port=5
  Vhcl.Wheel.FR : Inport  Port=6
  Vhcl.Wheel.RL : Inport  Port=7
  Vhcl.Wheel.RR : Inport  Port=8
  Car.Hitch.FrcTrq : Inport  Port=9
  Vhcl.Fr1A : Inport  Port=10
  CarAndTrailerUpd : S-Function  FunctionName=CM_Sfun  Parameters='CarAndTrUpd'  SFunctionDeploymentMode=off  EnableBusSupport=off
  CreateBus Brake.IF.In : Subsystem
  Sync_Out : Outport  VectorParamsAs1DForOutWhenUnconnected=off
  Brake.IF.In : Outport  Port=2  VectorParamsAs1DForOutWhenUnconnected=off
  wires:
  Vhcl.Fr1A/1 -> CarAndTrailerUpd/10  "user vehicle only"
  Vhcl.Steering/1 -> CarAndTrailerUpd/2
  Vhcl.Motion/1 -> CarAndTrailerUpd/3
  Vhcl.PoI/1 -> CarAndTrailerUpd/4
  Vhcl.Wheel.FL/1 -> CarAndTrailerUpd/5
  Vhcl.Wheel.FR/1 -> CarAndTrailerUpd/6
  Car.Hitch.FrcTrq/1 -> CarAndTrailerUpd/9
  Vhcl.Wheel.RR/1 -> CarAndTrailerUpd/8
  Vhcl.Wheel.RL/1 -> CarAndTrailerUpd/7
  CarAndTrailerUpd/2 -> CreateBus Brake.IF.In/1(In)
  CreateBus Brake.IF.In/1(Out) -> Brake.IF.In/1
  CarAndTrailerUpd/1 -> Sync_Out/1
  Sync_In/1 -> CarAndTrailerUpd/1

== system generic_src/CarMaker/IPG Vehicle/CarAndTrailer/Forces ==
  Sync_In : Inport
  TireFL_In : Inport  Port=2
  TireFR_In : Inport  Port=3
  TireRL_In : Inport  Port=4
  TireRR_In : Inport  Port=5
  lSpring : Inport  Port=6
  vDamp : Inport  Port=7
  lStabi : Inport  Port=8
  lBuf : Inport  Port=9
  External Suspension Forces : Subsystem
  Suspension Forces : Subsystem
  Tires : Subsystem
  Vehicle Forces : Subsystem
  Sync_Out : Outport  VectorParamsAs1DForOutWhenUnconnected=off
  Car.Virtual : Outport  Port=2  VectorParamsAs1DForOutWhenUnconnected=off
  Car.Aero : Outport  Port=3  VectorParamsAs1DForOutWhenUnconnected=off
  Car.Load : Outport  Port=4  VectorParamsAs1DForOutWhenUnconnected=off
  TireFL_Out : Outport  Port=5  VectorParamsAs1DForOutWhenUnconnected=off
  TireFR_Out : Outport  Port=6  VectorParamsAs1DForOutWhenUnconnected=off
  TireRL_Out : Outport  Port=7  VectorParamsAs1DForOutWhenUnconnected=off
  TireRR_Out : Outport  Port=8  VectorParamsAs1DForOutWhenUnconnected=off
  wires:
  lBuf/1 -> External Suspension Forces/5(lBuf)
  lStabi/1 -> External Suspension Forces/4(lStabi)
  vDamp/1 -> External Suspension Forces/3(vDamp)
  Tires/4(TireRR_Out) -> TireRR_Out/1
  Tires/3(TireRL_Out) -> TireRL_Out/1
  Tires/2(TireFR_Out) -> TireFR_Out/1
  Tires/1(TireFL_Out) -> TireFL_Out/1
  TireRR_In/1 -> Tires/5(TireRR_In)
  TireRL_In/1 -> Tires/4(TireRL_In)
  TireFR_In/1 -> Tires/3(TireFR_In)
  TireFL_In/1 -> Tires/2(TireFL_In)
  Sync_In/1 -> External Suspension Forces/1(Sync_In), Tires/1(Sync_In), Vehicle Forces/1(Sync_In)
  Vehicle Forces/1(Sync_Out) -> ?
  Vehicle Forces/2(Car.Virtual) -> Car.Virtual/1
  Vehicle Forces/3(Car.Aero) -> Car.Aero/1
  Vehicle Forces/4(Car.Load) -> Car.Load/1
  lSpring/1 -> External Suspension Forces/2(lSpring)
  ? -> Sync_Out/1

== system generic_src/CarMaker/IPG Vehicle/CarAndTrailer/Kinematics ==
  Sync_In : Inport
  Steer.IF : Inport  Port=2
  Kinematics : S-Function  FunctionName=CM_Sfun  Parameters='Kinematics'  SFunctionDeploymentMode=off  EnableBusSupport=off
  Sync_Out : Outport  VectorParamsAs1DForOutWhenUnconnected=off
  TireFL_In : Outport  Port=2  VectorParamsAs1DForOutWhenUnconnected=off
  TireFR_In : Outport  Port=3  VectorParamsAs1DForOutWhenUnconnected=off
  TireRL_In : Outport  Port=4  VectorParamsAs1DForOutWhenUnconnected=off
  TireRR_In : Outport  Port=5  VectorParamsAs1DForOutWhenUnconnected=off
  lSpring : Outport  Port=6  VectorParamsAs1DForOutWhenUnconnected=off
  vDamp : Outport  Port=7  VectorParamsAs1DForOutWhenUnconnected=off
  lStabi : Outport  Port=8  VectorParamsAs1DForOutWhenUnconnected=off
  lBuf : Outport  Port=9  VectorParamsAs1DForOutWhenUnconnected=off
  tWheelCarrier_z : Outport  Port=10  VectorParamsAs1DForOutWhenUnconnected=off
  wires:
  Steer.IF/1 -> Kinematics/2
  Kinematics/4 -> TireRL_In/1
  Kinematics/1 -> Sync_Out/1
  Kinematics/10 -> tWheelCarrier_z/1
  Kinematics/2 -> TireFL_In/1
  Kinematics/6 -> lSpring/1
  Sync_In/1 -> Kinematics/1
  Kinematics/8 -> lStabi/1
  Kinematics/9 -> lBuf/1
  Kinematics/5 -> TireRR_In/1
  Kinematics/3 -> TireFR_In/1
  Kinematics/7 -> vDamp/1

== system generic_src/CarMaker/IPG Vehicle/CarAndTrailer/Kinetics ==
  Sync_In : Inport
  Car.Virtual : Inport  Port=2
  Car.Aero : Inport  Port=3
  Car.Load : Inport  Port=4
  TireFL.Out : Inport  Port=5
  TireFR.Out : Inport  Port=6
  TireRL.Out : Inport  Port=7
  TireRR.Out : Inport  Port=8
  Bus Creator : BusCreator  Inputs=4
  Bus Creator1 : BusCreator  Inputs=12
  Bus Creator2 : BusCreator  Inputs=6
  Bus Creator3 : BusCreator  Inputs=6
  Bus Creator4 : BusCreator  Inputs=4
  Demux : Demux  Outputs=12
      settings: DisplayOption=none
  Demux1 : Demux  Outputs=6
      settings: DisplayOption=none
  Demux2 : Demux  Outputs=6
      settings: DisplayOption=none
  Demux3 : Demux
      settings: DisplayOption=none
  Demux4 : Demux
      settings: DisplayOption=none
  Kinetics : S-Function  FunctionName=CM_Sfun  Parameters='Kinetics'  SFunctionDeploymentMode=off  EnableBusSupport=off
  Sync_Out : Outport  VectorParamsAs1DForOutWhenUnconnected=off
  Trailer.Load : Outport  Port=2  VectorParamsAs1DForOutWhenUnconnected=off
  Car.Hitch : Outport  Port=3  VectorParamsAs1DForOutWhenUnconnected=off
  Car.Fr1 : Outport  Port=4  VectorParamsAs1DForOutWhenUnconnected=off
  Car.Trq_T2W : Outport  Port=5  VectorParamsAs1DForOutWhenUnconnected=off
  WheelCarrier.Misc : Outport  Port=6  VectorParamsAs1DForOutWhenUnconnected=off
  wires:
  Bus Creator1/1 -> Trailer.Load/1
  Demux/1 -> Bus Creator1/1  "Trailer Load_0 mass"
  Demux/2 -> Bus Creator1/2  "Trailer Load_0 tx"
  Demux/3 -> Bus Creator1/3  "Trailer Load_0 ty"
  Demux/4 -> Bus Creator1/4  "Trailer Load_0 tz"
  Demux/5 -> Bus Creator1/5  "Trailer Load_1 mass"
  Demux/6 -> Bus Creator1/6  "Trailer Load_1 tx"
  Demux/7 -> Bus Creator1/7  "Trailer Load_1 ty"
  Demux/8 -> Bus Creator1/8  "Trailer Load_1 tz"
  Demux/9 -> Bus Creator1/9  "Trailer Load_2 mass"
  Demux/10 -> Bus Creator1/10  "Trailer Load_2 tx"
  Demux/11 -> Bus Creator1/11  "Trailer Load_2 ty"
  Demux/12 -> Bus Creator1/12  "Trailer Load_2 tz"
  Demux1/1 -> Bus Creator2/1  "Car Hitch tx"
  Demux1/2 -> Bus Creator2/2  "Car Hitch ty"
  Demux1/3 -> Bus Creator2/3  "Car Hitch tz"
  Demux1/4 -> Bus Creator2/4  "Car Hitch vx"
  Demux1/5 -> Bus Creator2/5  "Car Hitch vy"
  Demux1/6 -> Bus Creator2/6  "Car Hitch vz"
  Bus Creator2/1 -> Car.Hitch/1
  Demux2/1 -> Bus Creator3/1  "Car Fr1 rx"
  Demux2/2 -> Bus Creator3/2  "Car Fr1 ry"
  Demux2/3 -> Bus Creator3/3  "Car Fr1 rz"
  Demux2/4 -> Bus Creator3/4  "Car Fr1 rvx"
  Demux2/5 -> Bus Creator3/5  "Car Fr1 rvy"
  Demux2/6 -> Bus Creator3/6  "Car Fr1 rvz"
  Bus Creator3/1 -> Car.Fr1/1
  Demux3/1 -> Bus Creator4/1  "car Susp FL GenInert2"
  Demux3/2 -> Bus Creator4/2  "car Susp FR GenInert2"
  Demux3/3 -> Bus Creator4/3  "car Susp FL GenFrc2"
  Demux3/4 -> Bus Creator4/4  "car Susp FR GenFrc2"
  Bus Creator4/1 -> WheelCarrier.Misc/1
  Bus Creator/1 -> Car.Trq_T2W/1
  Demux4/4 -> Bus Creator/4  "Car Trq_T2WRR"
  Demux4/3 -> Bus Creator/3  "Car Trq_T2WRL"
  Demux4/2 -> Bus Creator/2  "Car Trq_T2WFR"
  Demux4/1 -> Bus Creator/1  "Car Trq_T2WFL"
  Car.Aero/1 -> Kinetics/3
  Car.Load/1 -> Kinetics/4
  Car.Virtual/1 -> Kinetics/2
  TireRR.Out/1 -> Kinetics/8
  Kinetics/1 -> Sync_Out/1
  TireRL.Out/1 -> Kinetics/7
  Sync_In/1 -> Kinetics/1
  Kinetics/5 -> Demux4/1
  Kinetics/4 -> Demux2/1
  TireFL.Out/1 -> Kinetics/5
  Kinetics/2 -> Demux/1
  Kinetics/6 -> Demux3/1
  Kinetics/3 -> Demux1/1
  TireFR.Out/1 -> Kinetics/6

== system generic_src/CarMaker/IPG Vehicle/CarAndTrailer/Steering ==
  note: When replacing the entire steering system,
      | be sure to disable the IPG steering model by using the steering
      | model 'Model Manager off' in the vehicle GUI.
  Sync_In : Inport
  VhclCtrl.Steering : Inport  Port=2
  Bus Creator1 : BusCreator  Inputs=16
  Bus Creator2 : BusCreator  Inputs=5
  Demux : Demux  Outputs=21
      settings: DisplayOption=none
  Steering : S-Function  FunctionName=CM_Sfun  Parameters='Steering'  SFunctionDeploymentMode=off  EnableBusSupport=off
  Terminator : Terminator
  Sync_Out : Outport  VectorParamsAs1DForOutWhenUnconnected=off
  Steer.IF : Outport  Port=2  VectorParamsAs1DForOutWhenUnconnected=off
  wires:
  Demux/21 -> Bus Creator2/5  "Steering IF R Inert"
  Demux/20 -> Bus Creator2/4  "Steering IF R Frc"
  Demux/19 -> Bus Creator2/3  "Steering IF L Inert"
  Demux/18 -> Bus Creator2/2  "Steering IF L Frc"
  Demux/17 -> Bus Creator2/1  "Steering IF SteerByTrq"
  Demux/16 -> Bus Creator1/16  "Steering IF R iSteer2q"
  Demux/15 -> Bus Creator1/15  "Steering IF R qpp"
  Demux/14 -> Bus Creator1/14  "Steering IF R qp"
  Demux/13 -> Bus Creator1/13  "Steering IF R q"
  Demux/12 -> Bus Creator1/12  "Steering IF L iSteer2q"
  Demux/11 -> Bus Creator1/11  "Steering IF L qpp"
  Demux/10 -> Bus Creator1/10  "Steering IF L qp"
  Demux/9 -> Bus Creator1/9  "Steering IF L q"
  Demux/8 -> Bus Creator1/8  "Steering IF AssistTrqPin"
  Demux/7 -> Bus Creator1/7  "Steering IF AssistTrqCol"
  Demux/6 -> Bus Creator1/6  "Steering IF AssistFrc"
  Demux/5 -> Bus Creator1/5  "Steering IF TrqStatic"
  Demux/4 -> Bus Creator1/4  "Steering IF Trq"
  Demux/3 -> Bus Creator1/3  "Steering IF AngAcc"
  Demux/2 -> Bus Creator1/2  "Steering IF AngVel"
  Demux/1 -> Bus Creator1/1  "Steering IF Ang"
  Bus Creator1/1 -> Steer.IF/1
  Steering/2 -> Demux/1
  Bus Creator2/1 -> Terminator/1  "Steer IF (in)"
  VhclCtrl.Steering/1 -> Steering/2
  Steering/1 -> Sync_Out/1
  Sync_In/1 -> Steering/1

== system generic_src/CarMaker/IPG Vehicle/CarAndTrailer/Trailer ==
  Sync_In : Inport
  Trailer.Load : Inport  Port=2
  Car.Hitch : Inport  Port=3
  Car.Fr1 : Inport  Port=4
  Car.Trq_T2W : Inport  Port=5
  WheelCarrier.Misc : Inport  Port=6
  CreateBus Car.Hitch.FrcTrq : Subsystem
  CreateBus Vhcl.Motion : Subsystem
  CreateBus Vhcl.PoI : Subsystem
  CreateBus Vhcl.Steering : Subsystem
  CreateBus Vhcl.Wheel.FL : Subsystem
  CreateBus Vhcl.Wheel.FR : Subsystem
  CreateBus Vhcl.Wheel.RL : Subsystem
  CreateBus Vhcl.Wheel.RR : Subsystem
  Trailer : S-Function  FunctionName=CM_Sfun  Parameters='Trailer'  SFunctionDeploymentMode=off  EnableBusSupport=off
  Sync_Out : Outport  VectorParamsAs1DForOutWhenUnconnected=off
  Vhcl.Steering : Outport  Port=2  VectorParamsAs1DForOutWhenUnconnected=off
  Vhcl.Motion : Outport  Port=3  VectorParamsAs1DForOutWhenUnconnected=off
  Vhcl.PoI : Outport  Port=4  VectorParamsAs1DForOutWhenUnconnected=off
  Vhcl.Wheel.FL : Outport  Port=5  VectorParamsAs1DForOutWhenUnconnected=off
  Vhcl.Wheel.FR : Outport  Port=6  VectorParamsAs1DForOutWhenUnconnected=off
  Vhcl.Wheel.RL : Outport  Port=7  VectorParamsAs1DForOutWhenUnconnected=off
  Vhcl.Wheel.RR : Outport  Port=8  VectorParamsAs1DForOutWhenUnconnected=off
  Car.Hitch.FrcTrq : Outport  Port=9  VectorParamsAs1DForOutWhenUnconnected=off
  wires:
  Trailer/2 -> CreateBus Vhcl.Steering/1(In1)
  CreateBus Vhcl.Steering/1(Out1) -> Vhcl.Steering/1  "Vhcl.Steering"
  Trailer/3 -> CreateBus Vhcl.Motion/1(In1)
  Trailer/4 -> CreateBus Vhcl.PoI/1(In1)
  Trailer/5 -> CreateBus Vhcl.Wheel.FL/1(In1)
  Trailer/6 -> CreateBus Vhcl.Wheel.FR/1(In1)
  Trailer/7 -> CreateBus Vhcl.Wheel.RL/1(In1)
  Trailer/9 -> CreateBus Car.Hitch.FrcTrq/1(In1)
  Trailer/8 -> CreateBus Vhcl.Wheel.RR/1(In1)
  CreateBus Vhcl.Wheel.RR/1(Out1) -> Vhcl.Wheel.RR/1  "Vhcl.Wheel.RR"
  CreateBus Vhcl.Wheel.RL/1(Out1) -> Vhcl.Wheel.RL/1  "Vhcl.Wheel.RL"
  CreateBus Vhcl.Wheel.FR/1(Out1) -> Vhcl.Wheel.FR/1  "Vhcl.Wheel.FR"
  CreateBus Vhcl.Wheel.FL/1(Out1) -> Vhcl.Wheel.FL/1  "Vhcl.Wheel.FL"
  CreateBus Vhcl.PoI/1(Out1) -> Vhcl.PoI/1  "Vhcl.PoI"
  CreateBus Vhcl.Motion/1(Out1) -> Vhcl.Motion/1  "Vhcl.Motion"
  Car.Trq_T2W/1 -> Trailer/5
  WheelCarrier.Misc/1 -> Trailer/6
  CreateBus Car.Hitch.FrcTrq/1(Out1) -> Car.Hitch.FrcTrq/1  "Car.Hitch.FrcTrq"
  Car.Fr1/1 -> Trailer/4
  Car.Hitch/1 -> Trailer/3
  Trailer.Load/1 -> Trailer/2
  Trailer/1 -> Sync_Out/1
  Sync_In/1 -> Trailer/1

== system generic_src/CarMaker/IPG Vehicle/PowerTrain/MCU Example ==
  Sync_In : Inport
  Bus Assignment : BusAssignment  AssignedSignals=MCU ISGOut Load,MCU ISGOut TrqMot_max,MCU ISGOut TrqGen_max
  Bus Creator : BusCreator  Inputs=5
  Bus Creator1 : BusCreator  Inputs=2
  Bus Creator2 : BusCreator  Inputs=2
  Bus Selector : BusSelector  OutputSignals=MCU Ignition,MCU ISGIn.MCU ISGIn rotv,MCU ISGIn.MCU ISGIn Trq_trg,MCU ISGOut.MCU ISGIn Load,MCU ISGIn.MCU ISGIn rotv_trg,MCU_Cfg ISG.MCU_Cfg ISG Ratio,MCU_Cfg ISG.MCU_Cfg ISG rotv_Mot_max,MCU_Cfg ISG.MCU_Cfg ISG rotv_Gen_max
  Constant : Constant  Value=xData
  Constant1 : Constant  Value=yData
  CreateBus MCU ISGOut : Subsystem
  CreateBus MCU MotorOut0 : Subsystem
  CreateBus MCU MotorOut1 : Subsystem
  CreateBus MCU MotorOut2 : Subsystem
  CreateBus MCU MotorOut3 : Subsystem
  CreateBus MCU Status : Subsystem
  Ground MCU ISGOut : Ground
  Ground MCU MotorOut{0..3} (4 alike) : Ground
  Ground MCU Status : Ground
  MyMotorCU : Subsystem
  PTMotorCU_In : Subsystem
  PTMotorCU_Out : Subsystem
  wires:
  Bus Assignment/1 -> PTMotorCU_Out/2(MCU ISGOut)
  CreateBus MCU ISGOut/1(Out) -> Bus Assignment/1
  Ground MCU ISGOut/1 -> CreateBus MCU ISGOut/1(In)
  MyMotorCU/3(TrqGen_max) -> Bus Assignment/4
  MyMotorCU/2(TrqMot_max) -> Bus Assignment/3
  MyMotorCU/1(Load out) -> Bus Assignment/2
  Constant1/1 -> Bus Creator2/2, Bus Creator1/2  "z"
  Constant/1 -> Bus Creator2/1, Bus Creator1/1  "x"
  Bus Creator2/1 -> Bus Creator/5  "TrqGen_max"
  Bus Selector/1 -> MyMotorCU/1(Ignition)  "<MCU Ignition>"
  PTMotorCU_In/1(PTMotorCU_In) -> Bus Selector/1
  Sync_In/1 -> PTMotorCU_In/1(Sync_In)
  Bus Selector/5 -> MyMotorCU/5(rotv_trg)  "<MCU ISGIn rotv_trg>"
  Bus Selector/4 -> MyMotorCU/4(Load)  "<MCU ISGIn Load>"
  Bus Selector/8 -> Bus Creator/3  "<MCU_Cfg ISG rotv_Gen_max>"
  Bus Selector/7 -> Bus Creator/2  "<MCU_Cfg ISG rotv_Mot_max>"
  Bus Creator1/1 -> Bus Creator/4  "TrqMot_max"
  Bus Selector/6 -> Bus Creator/1  "<MCU_Cfg ISG Ratio>"
  Bus Creator/1 -> MyMotorCU/6(CfgIF)
  Bus Selector/3 -> MyMotorCU/3(Trq_trg)  "<MCU ISGIn Trq_trg>"
  Bus Selector/2 -> MyMotorCU/2(rotv)  "<MCU ISGIn rotv>"
  CreateBus MCU MotorOut3/1(Out) -> PTMotorCU_Out/6(MCU MotorOut3)
  Ground MCU MotorOut3/1 -> CreateBus MCU MotorOut3/1(In)
  CreateBus MCU MotorOut2/1(Out) -> PTMotorCU_Out/5(MCU MotorOut2)
  Ground MCU MotorOut2/1 -> CreateBus MCU MotorOut2/1(In)
  CreateBus MCU MotorOut1/1(Out) -> PTMotorCU_Out/4(MCU MotorOut1)
  Ground MCU MotorOut1/1 -> CreateBus MCU MotorOut1/1(In)
  CreateBus MCU MotorOut0/1(Out) -> PTMotorCU_Out/3(MCU MotorOut0)
  Ground MCU MotorOut0/1 -> CreateBus MCU MotorOut0/1(In)
  CreateBus MCU Status/1(Out) -> PTMotorCU_Out/1(MCU Status)
  Ground MCU Status/1 -> CreateBus MCU Status/1(In)

== system generic_src/CarMaker/IPG Vehicle/PowerTrain/PTControl Example ==
  Sync_In : Inport
  VhclCtrl.PT : Inport  Port=2
  CreateBus PTC BatteryHVOut : Subsystem
  CreateBus PTC BatteryLVOut : Subsystem
  CreateBus PTC EngineOut : Subsystem
  CreateBus PTC ISGOut : Subsystem
  CreateBus PTC MiscOut : Subsystem
  CreateBus PTC PwrSupplyOut : Subsystem
  CreateBus PTC WheelOut : Subsystem
  Ground PTC PwrSupplyOut : Ground
  Ground PTC PwrSupplyOut1 : Ground
  Ground PTC PwrSupplyOut2 : Ground
  Ground PTC WheelOut : Ground
  PTC ClutchOut : Subsystem
  PTC GearBoxOut : Subsystem
  PTC MotorOut : Subsystem
  PTControl Example : Subsystem
  PTControl_In : Subsystem
  PTControl_Out : Subsystem
  wires:
  Sync_In/1 -> PTControl_In/1(Sync_In)
  VhclCtrl.PT/1 -> PTControl Example/2(VhclCtrl.PT)
  CreateBus PTC MiscOut/1(Out) -> PTControl_Out/1(PTC MiscOut)
  CreateBus PTC EngineOut/1(Out) -> PTControl_Out/2(PTC EngineOut)
  CreateBus PTC ISGOut/1(Out) -> PTControl_Out/3(PTC ISGOut)
  Ground PTC PwrSupplyOut/1 -> CreateBus PTC PwrSupplyOut/1(In)
  CreateBus PTC PwrSupplyOut/1(Out) -> PTControl_Out/7(PTC PwrSupplyOut)
  Ground PTC WheelOut/1 -> CreateBus PTC WheelOut/1(In)
  CreateBus PTC WheelOut/1(Out) -> PTControl_Out/10(PTC WheelOut)
  PTC ClutchOut/1(PTC ClutchOut) -> PTControl_Out/5(PTC ClutchOut)
  PTControl Example/3(ISGOut) -> CreateBus PTC ISGOut/1(In)
  PTControl Example/2(EngineOut) -> CreateBus PTC EngineOut/1(In)
  PTControl Example/1(PTC MiscOut) -> CreateBus PTC MiscOut/1(In)
  PTControl_In/1(PTControl_In) -> PTControl Example/1(EngineIn)
  Ground PTC PwrSupplyOut1/1 -> CreateBus PTC BatteryLVOut/1(In)
  Ground PTC PwrSupplyOut2/1 -> CreateBus PTC BatteryHVOut/1(In)
  CreateBus PTC BatteryLVOut/1(Out) -> PTControl_Out/8(PTC BattLV_Out)
  CreateBus PTC BatteryHVOut/1(Out) -> PTControl_Out/9(PTC BattHV_Out)
  PTC MotorOut/1(PTC MotorOut) -> PTControl_Out/4(PTC MotorOut)
  PTControl Example/4(ClutchOut Pos) -> PTC ClutchOut/1(ClutchOut Pos)
  PTControl Example/5(GearBoxOut GearNoTrg) -> PTC GearBoxOut/1(GearBoxOut GearNoTrg)
  PTC GearBoxOut/1(PTC GearboxOut) -> PTControl_Out/6(PTC GearboxOut)
